simulink model "solar"  (R2024b)
settings: Solver=VariableStepAuto  StartTime=0.0  StopTime=1  RelTol=1e-3
libraries: spsCurrentMeasurementLib x1, spsDiodeLib x1, spsPVArrayLib x1, spsSeriesRLCBranchLib x1, spsVoltageMeasurementLib x1, sps_lib x1
settings Model: Creator=SHRUTHI  LastModifiedBy=Mahesh

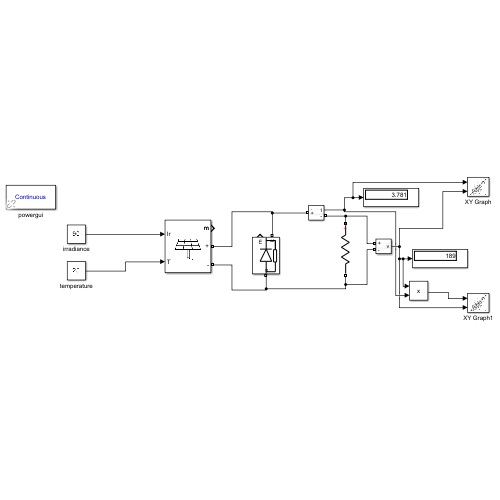
[thumbnail: Simulink's stored preview of the top-level diagram]
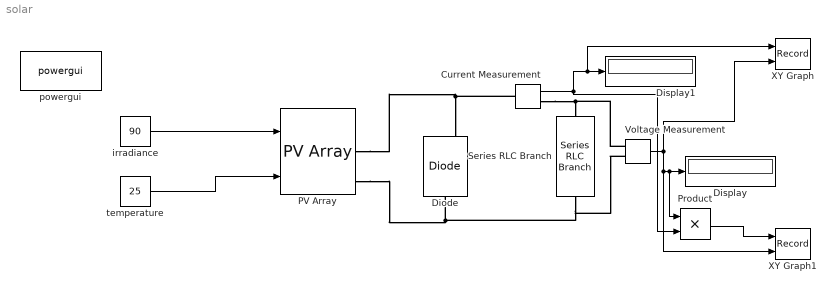
== system solar ==
  Current Measurement : spsCurrentMeasurementLib/Current Measurement  PhasorSimulation=off  OutputType=Complex  PSBequivalent=0
  Diode : spsDiodeLib/Diode  Ron=0.001  Lon=0  Vf=0.8  IC=0  UseSnubber=0  Rs=500  Cs=250e-9  Measurements=on
  Display : Display
  Display1 : Display
  PV Array : spsPVArrayLib/PV Array  Npar=40  Nser=10  PlotType=array @ 25 deg.C & specified irradiances  S_vec=[ 90 70 40 ]  Temp_C_vec="[ 45 25  ]"  ModuleName=User-defined  PlotWhenSelected=off  Pm=100.224  Ncell=60  Voc=21.40  Isc=6.41  Vm=17.4  Im=5.76  beta_Voc_pc=-0.41  alpha_Isc_pc=0.102  beta_Voc=-0.08774  alpha_Isc=0.0065382  IL=6.4049  I0=1.1462e-09  nI=0.62017  Rsh=58.1543  Rs=0.20876  RobustModel=off  RobustCellTemperature=313.3991  BAL=on  Tc=1e-6  Tfilter=5e-5
  Product : Product
  Series RLC Branch : spsSeriesRLCBranchLib/Series RLC Branch  LConnTagsString=__new0  RConnTagsString=__new0  BranchType=R  Resistance=50  Inductance=1e-3  SetiL0=off  InitialCurrent=0  Capacitance=1e-6  Setx0=off  InitialVoltage=0  Measurements=None
  Voltage Measurement : spsVoltageMeasurementLib/Voltage Measurement  PhasorSimulation=off  OutputType=Complex  PSBequivalent=0
  XY Graph : Record  FileSettingsInternal="{\"entries\":[{\"content\":{\"excelSettings\":{\"content\":{},\"type\":\"Streamout.ExcelSettings\"}},\"type\":\"Streamout.FileSettingStorage\",\"uuid\":\"\"}],\"packageUris\":[\"http:\\/\\/schema.mathworks.com\\/mf0\\/streamout_blocks\\/R2020a\"],\"version\":\"1.0\"}"  Layout=[1 1]  SignalsInternal="{\"entries\":[{\"content\":{\"signals\":[{\"content\":{\"blockPath\":[],\"dimensions\":[1],\"domain\":\"\",\"lineColor\":\"#a2142f\",\"plots\":[ 1 ],\"port\":1,\"sid\":[\"\"],\"signalID\":1,\"signalName\":\"Current Measurement\"},\"type\":\"RecordBlkView.Signal\",\"uuid\":\"\"},{\"content\":{\"blockPath\":[],\"dimensions\":[1],\"domain\":\"\",\"lineColor\":\"#139fff\",\"plots\":[ 1 ],\"port\":2,\"sid\":[\"\"],\"signalID\":2,\"signalName\":\"Voltage Measurement\"},\"type\":\"RecordBlkView.Signal\",\"uuid\":\"\"}]},\"type\":\"RecordBlkView.InputSignals\",\"uuid\":\"\"}],\"packageUris\":[\"http:\\/\\/schema.mathworks.com\\/mf0\\/streamout_blocks\\/R2020a\"],\"version\":\"1.0\"}"  VisualizationBindings="{\"xyplotplugin\":{\"info\":[{\"series\":[{\"bindingParametersList\":[{\"parameter\":\"X-Axis\",\"signalID\":2,\"signalName\":\"Voltage Measurement\"},{\"parameter\":\"Y-Axis\",\"signalID\":1,\"signalName\":\"Current Measurement\"}],\"seriesID\":0}],\"subplotID\":1}]}}"  CompatibilityTag=XY
  XY Graph1 : Record  FileSettingsInternal="{\"entries\":[{\"content\":{\"excelSettings\":{\"content\":{},\"type\":\"Streamout.ExcelSettings\"}},\"type\":\"Streamout.FileSettingStorage\",\"uuid\":\"\"}],\"packageUris\":[\"http:\\/\\/schema.mathworks.com\\/mf0\\/streamout_blocks\\/R2020a\"],\"version\":\"1.0\"}"  Layout=[1 1]  SignalsInternal="{\"entries\":[{\"content\":{\"signals\":[{\"content\":{\"blockPath\":[],\"dimensions\":[1],\"domain\":\"\",\"lineColor\":\"#a2142f\",\"plots\":[ 1 ],\"port\":1,\"sid\":[\"\"],\"signalID\":1,\"signalName\":\"Product\"},\"type\":\"RecordBlkView.Signal\",\"uuid\":\"\"},{\"content\":{\"blockPath\":[],\"dimensions\":[1],\"domain\":\"\",\"lineColor\":\"#139fff\",\"plots\":[ 1 ],\"port\":2,\"sid\":[\"\"],\"signalID\":2,\"signalName\":\"Voltage Measurement\"},\"type\":\"RecordBlkView.Signal\",\"uuid\":\"\"}]},\"type\":\"RecordBlkView.InputSignals\",\"uuid\":\"\"}],\"packageUris\":[\"http:\\/\\/schema.mathworks.com\\/mf0\\/streamout_blocks\\/R2020a\"],\"version\":\"1.0\"}"  VisualizationBindings="{\"xyplotplugin\":{\"info\":[{\"series\":[{\"bindingParametersList\":[{\"parameter\":\"X-Axis\",\"signalID\":2,\"signalName\":\"Voltage Measurement\"},{\"parameter\":\"Y-Axis\",\"signalID\":1,\"signalName\":\"Product\"}],\"seriesID\":0}],\"subplotID\":1}]}}"  CompatibilityTag=XY
  irradiance : Constant  Value=90
  powergui : sps_lib/powergui  Priority=1  SimulationMode=Continuous  SampleTime=50e-6  frequency=60  Iterations=50  frequencyindice=0  Pbase=100e6  ErrMax=1e-4  UnitsV=kV  UnitsW=MW  buscounter=0  FunctionMessages=off  echomessages=off  EnableUseOfTLC=off  CurrentSourceSwitches=off  DisableSnubberDevices=off  DisableRonSwitches=off  DisableVfSwitches=off  DisplayEquations=off  AutomaticDiscreteSolvers=off  SolverType=Tustin/Backward Euler (TBE)  Interpol=off  ExternalGateDelay=off  methode=off  Ts=100  x0status=blocks  SPID=on  SwTol=0  HookPort=off  NonlinearTolerance=1e-4  nMaxIteration=100  ContinueOnMaxIteration=off  RestoreLinks=warning  ResistiveCurrentMeasurement=off  Frange=[0:2:500]  Ylog=off  Xlog=on  ShowGrid=off  save=off  variable=ZData  structure=0  ZoomFFT=off  StartTime=0.0  cycles=1  DisplayStyle=1  fundamental=60  FreqAxis=off  MaxFrequency=1000  frequencyindicesteady=1  RmsSteady=1  display=off
  temperature : Constant  Value=25
  wires:
  irradiance/1 -> PV Array/1
  temperature/1 -> PV Array/2
  Voltage Measurement/1 -> XY Graph1/2, Product/1, Display/1, XY Graph/2
  Current Measurement/1 -> XY Graph/1, Display1/1, Product/2
  Product/1 -> XY Graph1/1
  connections:
  PV Array/RConn1 -- Diode/RConn1 -- Current Measurement/LConn1
  PV Array/RConn2 -- Voltage Measurement/LConn2 -- Series RLC Branch/RConn1 -- Diode/LConn1
  Current Measurement/RConn1 -- Voltage Measurement/LConn1 -- Series RLC Branch/LConn1
